simulink library "AFCToolbox2023a"  (R2023a)
settings: Solver=VariableStepAuto  StartTime=0.0  StopTime=10.0  RelTol=1e-3
undefined symbols (not defined in the file or in its folder): AFC5Toolbox_SimuMoudle, AFCToolbox, ax, ay, az, btnSample, C_d, C_dm, C_m, C_t, Control, d, declination_table, dp0, dp1, dp2, dp3, dt, euler_0, g0, I_xyz, inclination_table, J_m, lmd_high, lmd_low, lp_acc_knoise, lp_acc_max, lp_acc_min, lp_acc_seed, lp_GPS_BL_max, lp_GPS_BL_min, lp_GPS_H_max, lp_GPS_H_min, lp_GPS_knoise, lp_GPS_seed, lp_GPS_vel_max, lp_GPS_vel_min, lp_gyro_knoise, lp_gyro_max, lp_gyro_min, lp_gyro_seed, lp_hf_vwind, lp_hs_vwind_interp, lp_kaerorho, lp_kaeroT, lp_kIxyz, lp_kmass, lp_momentx_A0, lp_momentx_Af, lp_momentx_ts, lp_momenty_A0, lp_momenty_Af, lp_momenty_ts, lp_momentz_A0, lp_momentz_Af, lp_momentz_ts, lp_vf_vwind, lp_vs_vwind_interp, lp_vwind_thetax, lp_vwind_thetaz ... (+54)
libraries: $bdroot x104, simulink x75, etargetslib x32, sharedtransform x13, simulink_extras x12, dspstat3 x11, aerolibconvert2 x9, aerolibtransform2 x3, aerolibutil x2, matrix_library x1
(part 6 of 10)

== system AFCToolbox2023a/基础导航算法模型库/ECL EKF/init_state/LLA2NED ==
  note: Vecef2ned
  gps_LLA_rad : Inport
  GPSfixtype : Inport  Port=2
  GPS_Vecef_m/s : Inport  Port=3
  QGC_sensor_reinit : Inport  Port=4
  Angle Conversion1 : aerolibconvert2/Angle Conversion  IU=deg  OU=rad
  Bus Creator : BusCreator  Inputs=3
  Bus Creator2 : BusCreator  Inputs=3
  Bus Selector : BusSelector  OutputSignals=lon_gps,lat_gps
  Bus Selector1 : BusSelector  OutputSignals=lat_gps,lon_gps,H_gps
  Constant1 : Constant  Value=-90
  Constant4 : Constant  Value=0
  Data Type Conversion{,1..3} (4 alike) : DataTypeConversion  OutDataTypeStr=single  SaturateOnIntegerOverflow=off  RndMeth=Floor
  Demux : Demux  Outputs=3
  Demux1 : Demux  Outputs=3
  Demux3 : Demux  Outputs=3
  Detect Increase : simulink/Logic and Bit Operations/Detect Increase  vinit=0.0  OutDataTypeStr=boolean
  Direction Cosine Matrix ECEF to NED : aerolibtransform2/Direction Cosine Matrix ECEF to NED  Commented=on
  Display2 : Display
  Divide1 : Product  Inputs=**  Multiplication=Matrix(*)
  From Workspace22 : FromWorkspace  Commented=on  VariableName=[AFC5_Data.Tim,Pn]  SampleTime=0.01
  From Workspace23 : FromWorkspace  Commented=on  VariableName=[AFC5_Data.Tim,Pe]  SampleTime=0.01
  From Workspace24 : FromWorkspace  Commented=on  VariableName=[AFC5_Data.Tim,Pd]  SampleTime=0.01
  Gain : Gain  Gain=-1
  LLA to ECEF Position : LLA2ECEF  R=6378137
  LLA to ECEF Position1 : LLA2ECEF  R=6378137
  Mux2 : Mux  Inputs=3
  Mux3 : Mux  Commented=on  Inputs=3
  Mux5 : Mux  Inputs=2
  Mux6 : Mux  Inputs=2
  Product : Product  Commented=on  Multiplication=Matrix(*)
  Radians to Degrees{,1..3} (4 alike) : simulink_extras/Transformations/Radians to Degrees
  Radians to Degrees4 : simulink_extras/Transformations/Radians to Degrees  Commented=on
  Rotation Angles to Direction Cosine Matrix : sharedtransform/Rotation Angles to Direction Cosine Matrix  rotationOrder=ZYX  aMode=aMode
  Scope7 : Scope  NumInputPorts=2
  Selector2 : Selector  Commented=on  InputPortWidth=3  IndexOptions=Index vector (dialog)  Indices=[1 2]  OutputSizes=1
  Selector4 : Selector  InputPortWidth=3  IndexOptions=Index vector (dialog)  Indices=[3]  OutputSizes=1
  Sum : Sum  Inputs=|++
  Sum1 : Sum  Inputs=|+-
  initGPSLLA : MATLAB Function  TreatAsAtomicUnit=on
  gpsvNEDout : Outport
  "gpsposNEDout " : Outport  Port=2
  gps_alt_aef : Outport  Port=3
  wires:
  From Workspace24/1 -> Mux3/3
  From Workspace22/1 -> Mux3/1
  From Workspace23/1 -> Mux3/2
  Bus Creator2/1 -> "gpsposNEDout "/1  "data_Pned"
  GPSfixtype/1 -> initGPSLLA/2(GPSfixtype)
  Demux3/3 -> Data Type Conversion2/1  "gpspos_D"
  Demux3/2 -> Data Type Conversion1/1  "gpspos_E"
  Demux3/1 -> Data Type Conversion/1  "gpspos_N"
  Bus Creator/1 -> Bus Selector/1, Bus Selector1/1
  Demux/3 -> Bus Creator/3  "H_gps"
  Demux/2 -> Bus Creator/2  "lon_gps"
  Demux/1 -> Bus Creator/1  "lat_gps"
  Demux1/3 -> LLA to ECEF Position1/2
  Mux6/1 -> LLA to ECEF Position1/1
  Mux5/1 -> LLA to ECEF Position/1
  Gain/1 -> Sum/1
  LLA to ECEF Position1/1 -> Sum1/1
  Constant4/1 -> Mux2/3
  Sum1/1 -> Divide1/2
  Divide1/1 -> Demux3/1
  Demux1/1 -> Radians to Degrees/1
  Rotation Angles to Direction Cosine Matrix/1 -> Divide1/1
  Constant1/1 -> Angle Conversion1/1
  LLA to ECEF Position/1 -> Display2/1, Sum1/2, Selector4/1
  Demux1/2 -> Radians to Degrees1/1
  Sum/1 -> Mux2/2
  Bus Selector/2 -> Gain/1  "<lat_gps>"
  Bus Selector/1 -> Mux2/1  "<lon_gps>"
  Bus Selector1/1 -> Radians to Degrees2/1  "<lat_gps>"
  Bus Selector1/2 -> Radians to Degrees3/1  "<lon_gps>"
  Bus Selector1/3 -> LLA to ECEF Position/2  "<H_gps>"
  Radians to Degrees/1 -> Mux6/1
  Radians to Degrees1/1 -> Mux6/2
  QGC_sensor_reinit/1 -> Detect Increase/1
  Data Type Conversion/1 -> Bus Creator2/1  "gpspos_N"
  Data Type Conversion1/1 -> Bus Creator2/2  "gpspos_E"
  Angle Conversion1/1 -> Sum/2
  Radians to Degrees2/1 -> Mux5/1
  Radians to Degrees3/1 -> Mux5/2
  GPS_Vecef_m/s/1 -> Data Type Conversion3/1
  Direction Cosine Matrix ECEF to NED/1 -> Product/1
  Selector2/1 -> Radians to Degrees4/1
  Radians to Degrees4/1 -> Direction Cosine Matrix ECEF to NED/1
  Data Type Conversion3/1 -> gpsvNEDout/1
  Detect Increase/1 -> initGPSLLA/1(QGCinitflag)
  initGPSLLA/1(gpsLLA0_rad) -> Demux/1
  Selector4/1 -> Scope7/2
  Mux2/1 -> Rotation Angles to Direction Cosine Matrix/1
  gps_LLA_rad/1 -> Selector2/1, Demux1/1, initGPSLLA/3(gps_LLA_rad)
  Data Type Conversion2/1 -> Bus Creator2/3  "gpspos_D"

== system AFCToolbox2023a/基础导航算法模型库/ECL EKF/init_state/State_mag1 ==
  mag : Inport
  gps_LLA_rad : Inport  Port=2
  states : Inport  Port=3
  Atan2 : Trigonometry  Operator=atan2
  Bus Creator : BusCreator  Inputs=5
  Constant1 : Constant
  Constant2 : Constant  Value=0
  Data Type Conversion1 : DataTypeConversion  OutDataTypeStr=double  SaturateOnIntegerOverflow=off  RndMeth=Floor
  Data Type Conversion2 : DataTypeConversion  OutDataTypeStr=double  SaturateOnIntegerOverflow=off  RndMeth=Floor
  Data Type Conversion3 : DataTypeConversion  OutDataTypeStr=double  SaturateOnIntegerOverflow=off  RndMeth=Floor
  Demux : Demux  Outputs=3
  Demux2 : Demux  Outputs=3
  Detect Increase : simulink/Logic and Bit Operations/Detect Increase  vinit=0.0  OutDataTypeStr=boolean
  Digital Clock : DigitalClock  SampleTime=-1
  Display : Display
  Display1 : Display
  Display2 : Display
  Math Function2 : Math  Commented=on  Operator=transpose  SignedPower=on
  Memory : Memory  InheritSampleTime=on
  Mux2 : Mux  Inputs=3
  Quaternions to Direction Cosine Matrix : sharedtransform/Quaternions to  Direction Cosine Matrix  Commented=on  aMode=aMode
      settings: LibrarySourceBlock=|
      | aerolibtransform2/Quaternions to
      | Direction Cosine Matrix
  Radians to Degrees : simulink_extras/Transformations/Radians to Degrees
  Scope{1..6} (6 alike) : Scope
  Selector1 : Selector  Commented=on  InputPortWidth=24  IndexOptions=Index vector (dialog)  Indices=[1,2,3,4]  OutputSizes=1
  Subsystem : Subsystem
  Subsystem1 : Subsystem  Commented=on  mask{declination_table=declination_table, inclination_table=inclination_table, strength_table=strength_table}
      mask prompts: declination_table "Declination Lookup Table"; inclination_table "Magnitude Lookup Table"; strength_table "Inclination Lookup Table"
      mask DialogControl ParameterGroupVar Prompt: 参数
  Switch : Switch  Criteria=u2 > Threshold  SaturateOnIntegerOverflow=off  InputSameDT=off
  Switch2 : Switch  Threshold=1  SaturateOnIntegerOverflow=off  InputSameDT=off
  Terminator : Terminator
  Terminator1 : Terminator
  Zero-Order Hold : ZeroOrderHold  SampleTime=-1
  calculate_synthetic_mag_z_measurement : Subsystem  Commented=on
  initMag1 : MATLAB Function  Commented=on  TreatAsAtomicUnit=on
  mag_lpf : Subsystem
  init_MagB : Outport
  magdata : Outport  Port=2
  wires:
  Radians to Degrees/1 -> Scope6/1
  Atan2/1 -> Radians to Degrees/1
  Bus Creator/1 -> magdata/1
  gps_LLA_rad/1 -> Demux/1
  Demux/1 -> Scope2/1, Subsystem1/1(lat_rad)
  Demux/2 -> Subsystem1/2(lon_rad)
  Demux/3 -> Terminator/1
  Demux2/1 -> Mux2/1, Atan2/2
  mag/1 -> Scope5/1, Bus Creator/2, Demux2/1, calculate_synthetic_mag_z_measurement/1(measMag), Zero-Order Hold/1, Display1/1, mag_lpf/1(Mag_Data)  "measMag"
  Demux2/2 -> Mux2/2, Atan2/1
  Subsystem1/1(mag_declination_gps) -> Scope1/1, Data Type Conversion2/1  "mag_declination_gps"
  Subsystem1/2(mag_inclination_gps) -> Data Type Conversion1/1, Scope3/1  "mag_inclination_gps"
  Subsystem1/3(mag_strength_gps) -> Data Type Conversion3/1  "mag_strength_gps"
  calculate_synthetic_mag_z_measurement/1(mag_z_body_pred) -> Mux2/3
  Quaternions to Direction Cosine Matrix/1 -> Math Function2/1
  Demux2/3 -> Terminator1/1
  Data Type Conversion2/1 -> Display/1, calculate_synthetic_mag_z_measurement/2(_mag_declination_gps), Bus Creator/3  "mag_declination_gps"
  Data Type Conversion1/1 -> calculate_synthetic_mag_z_measurement/3(_mag_inclination_gps), Bus Creator/4  "mag_inclination_gps"
  Data Type Conversion3/1 -> calculate_synthetic_mag_z_measurement/4(_mag_strength_gps), Bus Creator/5  "mag_strength_gps"
  states/1 -> Selector1/1
  Selector1/1 -> Quaternions to Direction Cosine Matrix/1
  Constant2/1 -> Switch/3
  Digital Clock/1 -> Switch/2
  Constant1/1 -> Switch/1
  Switch/1 -> Detect Increase/1
  Detect Increase/1 -> Switch2/2
  Zero-Order Hold/1 -> Switch2/1, Memory/1, Display2/1, init_MagB/1, Bus Creator/1, Subsystem/1(data)  "init_MagB"
  Memory/1 -> Switch2/3

== system AFCToolbox2023a/SimuMoudle/Forces & Moments1/Moments/Disturb/Dist Mx ==
  N : Inport
  Step2 : Step  Time=ts_0  Before=A0  After=Af
  Sum : Sum  Inputs=|++
  D : Outport
  wires:
  Sum/1 -> D/1
  N/1 -> Sum/1
  Step2/1 -> Sum/2

== system AFCToolbox2023a/SimuMoudle/Forces & Moments1/Moments/Disturb/Dist My ==
  N : Inport
  Step2 : Step  Time=ts_0  Before=A0  After=Af
  Sum : Sum  Inputs=|++
  D : Outport
  wires:
  Step2/1 -> Sum/2
  N/1 -> Sum/1
  Sum/1 -> D/1

== system AFCToolbox2023a/SimuMoudle/Forces & Moments1/Moments/Disturb/Dist Mz ==
  N : Inport
  Step2 : Step  Time=ts_0  Before=A0  After=Af
  Sum : Sum  Inputs=|++
  D : Outport
  wires:
  Sum/1 -> D/1
  N/1 -> Sum/1
  Step2/1 -> Sum/2

== system AFCToolbox2023a/SimuMoudle/Forces & Moments1/Parameters/Air Parameter1/Air Model ==
  note: rho
  v : Inport
  h (km) : Inport  Port=2
  1/2 : Constant  Value=0.5
  Gain lp_kaeroT : Gain  Gain=lp_kaeroT
  Gain lp_kaerorho : Gain  Gain=lp_kaerorho
  H : Subsystem
      mask Display: disp('h --> H')
  Math Function : Math  Operator=sqrt  SignedPower=on
  Math Function1 : Math  Operator=pow  SignedPower=on
  Math Function2 : Math  Operator=pow  SignedPower=on
  PSL : Constant  Value=101325
  Pressure xishu : Subsystem
  Product : Product  Inputs=/*  SaturateOnIntegerOverflow=on  OutDataTypeStr=Inherit: Same as first input
  Product1 : Product  RndMeth=Zero
  Product2 : Product  Inputs=3  RndMeth=Zero
  Product3 : Product  Inputs=4  RndMeth=Zero
  Product4 : Product  Inputs=3  RndMeth=Zero
  T : Subsystem
  T xishu : Subsystem
  W : Subsystem
  W zhishu : Subsystem
  W zhishu1 : Subsystem
  constant2 : Constant  Value=20.0468
  rho xishu : Subsystem
  rhoSL : Constant  Value=1.225
  dongYaTou : Outport
  Mach : Outport  Port=2
  Pressure : Outport  Port=3
  wires:
  Product4/1 -> Pressure/1
  PSL/1 -> Product4/3
  Math Function2/1 -> Product4/1
  Pressure xishu/1(xishu) -> Product4/2
  W zhishu1/1(zhishu) -> Math Function2/2
  Gain lp_kaerorho/1 -> Product3/4
  Gain lp_kaeroT/1 -> Math Function/1
  v/1 -> Product3/1, Product/2, Product3/2
  Product/1 -> Mach/1
  Product1/1 -> Product/1
  1/2/1 -> Product3/3
  T/1(T) -> Gain lp_kaeroT/1
  h (km)/1 -> H/1(h), T/1(Z), Pressure xishu/1(Z), W zhishu1/1(Z), rho xishu/1(Z), W zhishu/1(Z), W/2(Z), T xishu/1(Z)
  H/1(H) -> Pressure xishu/2(H), W/1(H)
  W zhishu/1(zhishu) -> Math Function1/2
  Product3/1 -> dongYaTou/1
  Product2/1 -> Gain lp_kaerorho/1
  rhoSL/1 -> Product2/3
  rho xishu/1(xishu) -> Product2/2
  Math Function1/1 -> Product2/1
  W/1(W) -> Math Function2/1, Math Function1/1, T/3(W)
  T xishu/1(T xishu) -> T/2(T xishu)
  constant2/1 -> Product1/2
  Math Function/1 -> Product1/1

== system AFCToolbox2023a/SimuMoudle/Forces & Moments1/Parameters/Wind Velocity/Vector ==
  abs : Inport
  thetaz : Inport  Port=2
  thetax : Inport  Port=3
  Mux : Mux  Inputs=3
  Selector : Selector  InputPortWidth=3  IndexOptions=Index vector (dialog)  Indices=[3 2 1]  OutputSizes=1
  sin thetax cos thetax : Trigonometry  Operator=sincos
  sin thetaz cos thetaz : Trigonometry  Operator=sincos
  vwind cos z : Product  RndMeth=Zero
  vwind sin z : Product  RndMeth=Zero
  vwind xy cos x : Product  RndMeth=Zero
  vwind xy sin x : Product  RndMeth=Zero
  xyz : Outport
  wires:
  abs/1 -> vwind cos z/1, vwind sin z/1
  sin thetaz cos thetaz/1 -> vwind sin z/2
  sin thetaz cos thetaz/2 -> vwind cos z/2
  vwind sin z/1 -> Mux/1
  sin thetax cos thetax/1 -> vwind xy sin x/2
  sin thetax cos thetax/2 -> vwind xy cos x/2
  vwind cos z/1 -> vwind xy cos x/1, vwind xy sin x/1
  vwind xy cos x/1 -> Mux/3
  vwind xy sin x/1 -> Mux/2
  Mux/1 -> Selector/1
  thetaz/1 -> sin thetaz cos thetaz/1
  Selector/1 -> xyz/1
  thetax/1 -> sin thetax cos thetax/1

== system AFCToolbox2023a/SimuMoudle/Position-Control/Consistent formation control /一致性控制——F1/Subsystem1 ==
  Constant : Constant  Value=0.01
  MATLAB Function : MATLAB Function  TreatAsAtomicUnit=on
  Mux : Mux  Inputs=3
  Ramp : simulink/Sources/Ramp  slope=1  start=0  InitialOutput=0
  wxyz : Outport
  wires:
  Mux/1 -> wxyz/1
  MATLAB Function/2(wy) -> Mux/2, Mux/3
  MATLAB Function/1(wx) -> Mux/1
  Constant/1 -> MATLAB Function/2(dt)
  Ramp/1 -> MATLAB Function/1(i)

== system AFCToolbox2023a/SimuMoudle/Position-Control/Consistent formation control /一致性控制——F2/Subsystem2 ==
  Constant : Constant  Value=0.01
  MATLAB Function : MATLAB Function  TreatAsAtomicUnit=on
  Mux : Mux  Inputs=3
  Ramp : simulink/Sources/Ramp  slope=1  start=0  InitialOutput=0
  wxyz : Outport
  wires:
  Mux/1 -> wxyz/1
  MATLAB Function/2(wy) -> Mux/2, Mux/3
  MATLAB Function/1(wx) -> Mux/1
  Constant/1 -> MATLAB Function/2(dt)
  Ramp/1 -> MATLAB Function/1(i)

== system AFCToolbox2023a/SimuMoudle/Position-Control/Consistent formation control /一致性控制——F3/Subsystem1 ==
  Constant : Constant  Value=0.01
  MATLAB Function : MATLAB Function  TreatAsAtomicUnit=on
  Mux : Mux  Inputs=3
  Ramp : simulink/Sources/Ramp  slope=1  start=0  InitialOutput=0
  wxyz : Outport
  wires:
  Mux/1 -> wxyz/1
  MATLAB Function/2(wy) -> Mux/2, Mux/3
  MATLAB Function/1(wx) -> Mux/1
  Constant/1 -> MATLAB Function/2(dt)
  Ramp/1 -> MATLAB Function/1(i)

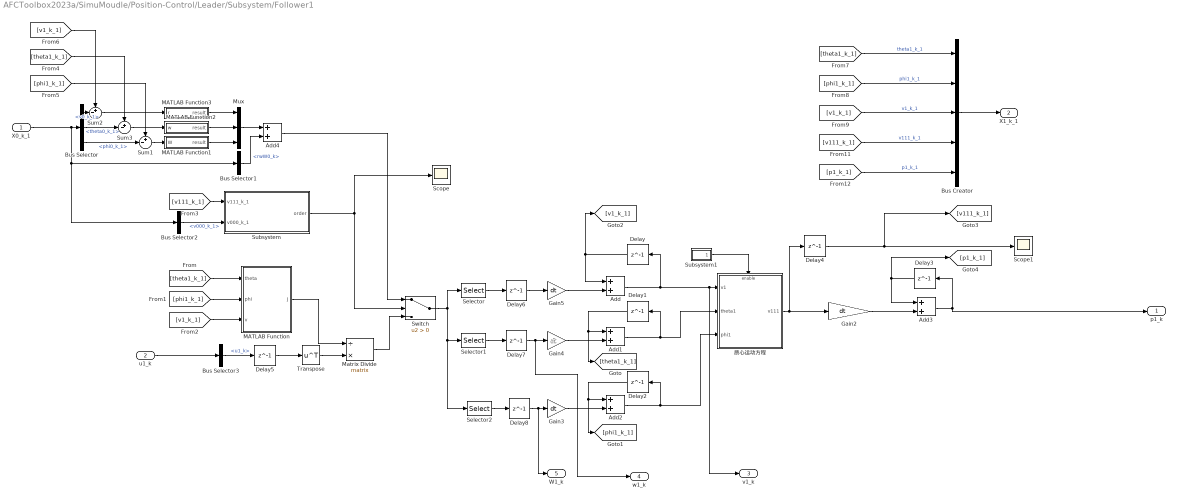
== system AFCToolbox2023a/SimuMoudle/Position-Control/Leader/Subsystem/Follower1 ==
  note: dt
  X0_k_1 : Inport
  u1_k : Inport  Port=2
  Add{,1..4} (5 alike) : Sum
  Bus Creator : BusCreator  Inputs=5
  Bus Selector : BusSelector  OutputSignals=v0_k_1,theta0_k_1,phi0_k_1
  Bus Selector1 : BusSelector  OutputSignals=rwW0_k
  Bus Selector2 : BusSelector  OutputSignals=v000_k_1
  Bus Selector3 : BusSelector  OutputSignals=u1_k
  Delay : Delay  DelayLength=1  InitialCondition=v1
  Delay1 : Delay  DelayLength=1  InitialCondition=theta1
  Delay2 : Delay  DelayLength=1  InitialCondition=phi1
  Delay3 : Delay  DelayLength=1  InitialCondition=p1
  Delay4 : Delay  DelayLength=1  InitialCondition=v111
  Delay5 : Delay  DelayLength=1  InitialCondition=u1
  Delay6 : Delay  DelayLength=1  InitialCondition=r1
  Delay7 : Delay  DelayLength=1  InitialCondition=w1
  Delay8 : Delay  DelayLength=1  InitialCondition=W1
  Gain{2..5} (4 alike) : Gain  Gain=dt
  MATLAB Function : MATLAB Function  TreatAsAtomicUnit=on
  MATLAB Function1 : MATLAB Function  TreatAsAtomicUnit=on
  MATLAB Function2 : MATLAB Function  TreatAsAtomicUnit=on
  MATLAB Function3 : MATLAB Function  TreatAsAtomicUnit=on
  Matrix Divide : Product  Inputs=/*  Multiplication=Matrix(*)
  Mux : Mux  Inputs=3
  Scope : Scope
  Scope1 : Scope
  Selector : Selector  InputPortWidth=3  IndexOptions=Index vector (dialog)  Indices=[1]  OutputSizes=1
  Selector1 : Selector  InputPortWidth=3  IndexOptions=Index vector (dialog)  Indices=[2]  OutputSizes=1
  Selector2 : Selector  InputPortWidth=3  IndexOptions=Index vector (dialog)  Indices=[3]  OutputSizes=1
  Subsystem : Subsystem
  Subsystem1 : Subsystem
  Sum1 : Sum  Inputs=+-|
  Sum2 : Sum  Inputs=+-|
  Sum3 : Sum  Inputs=+-|
  Switch : Switch  Criteria=u2 > Threshold  SaturateOnIntegerOverflow=off  InputSameDT=off
  Transpose : Math  Operator=transpose
  质心运动方程 : Subsystem
  p1_k : Outport
  X1_k_1 : Outport  Port=2
  v1_k : Outport  Port=3
  w1_k : Outport  Port=4
  W1_k : Outport  Port=5
  wires:
  Subsystem1/1(Out1) -> 质心运动方程/Enable
  Add3/1 -> Delay3/1, p1_k/1
  Delay1/1 -> Add1/1, [theta1_k_1]
  Transpose/1 -> Matrix Divide/2
  Bus Selector3/1 -> Delay5/1  "<u1_k>"
  Delay4/1 -> Scope1/1, [v111_k_1]
  Delay8/1 -> Gain3/1, W1_k/1
  Delay7/1 -> Gain4/1, w1_k/1
  Delay6/1 -> Gain5/1
  Add4/1 -> Switch/1
  Delay5/1 -> Transpose/1
  [theta1_k_1] -> Bus Creator/1  "theta1_k_1"
  [phi1_k_1] -> Bus Creator/2  "phi1_k_1"
  Bus Creator/1 -> X1_k_1/1
  [v1_k_1] -> Bus Creator/3  "v1_k_1"
  [p1_k_1] -> Bus Creator/5  "p1_k_1"
  [v111_k_1] -> Bus Creator/4  "v111_k_1"
  [v1_k_1] -> Sum2/1
  [phi1_k_1] -> Sum1/1
  [theta1_k_1] -> Sum3/1
  Sum1/1 -> MATLAB Function1/1(W)
  Sum2/1 -> MATLAB Function3/1(r)
  Bus Selector/1 -> Sum2/2  "<v0_k_1>"
  Bus Selector/3 -> Sum1/2  "<phi0_k_1>"
  Sum3/1 -> MATLAB Function2/1(w)
  Bus Selector/2 -> Sum3/2  "<theta0_k_1>"
  Mux/1 -> Add4/1
  MATLAB Function3/1(result) -> Mux/1
  MATLAB Function1/1(result) -> Mux/3
  MATLAB Function2/1(result) -> Mux/2
  Bus Selector1/1 -> Add4/2  "<rwW0_k>"
  X0_k_1/1 -> Bus Selector/1, Bus Selector1/1, Bus Selector2/1
  Bus Selector2/1 -> Subsystem/2(v000_k_1)  "<v000_k_1>"
  [v111_k_1] -> Subsystem/1(v111_k_1)
  质心运动方程/1(v111) -> Gain2/1, Delay4/1
  Matrix Divide/1 -> Switch/3
  Subsystem/1(order) -> Scope/1, Switch/2
  Selector2/1 -> Delay8/1
  Selector1/1 -> Delay7/1
  Selector/1 -> Delay6/1
  u1_k/1 -> Bus Selector3/1
  MATLAB Function/1(J) -> Matrix Divide/1
  Gain5/1 -> Add/2
  Add/1 -> Delay/1, 质心运动方程/1(v1), v1_k/1
  Delay/1 -> [v1_k_1], Add/1
  Add1/1 -> Delay1/1, 质心运动方程/2(theta1)
  Add2/1 -> Delay2/1, 质心运动方程/3(phi1)
  Delay2/1 -> Add2/1, [phi1_k_1]
  Gain2/1 -> Add3/2
  Delay3/1 -> [p1_k_1], Add3/1
  Switch/1 -> Selector/1, Selector1/1, Selector2/1
  Gain3/1 -> Add2/2
  Gain4/1 -> Add1/2
  [theta1_k_1] -> MATLAB Function/1(theta)
  [phi1_k_1] -> MATLAB Function/2(phi)
  [v1_k_1] -> MATLAB Function/3(v)

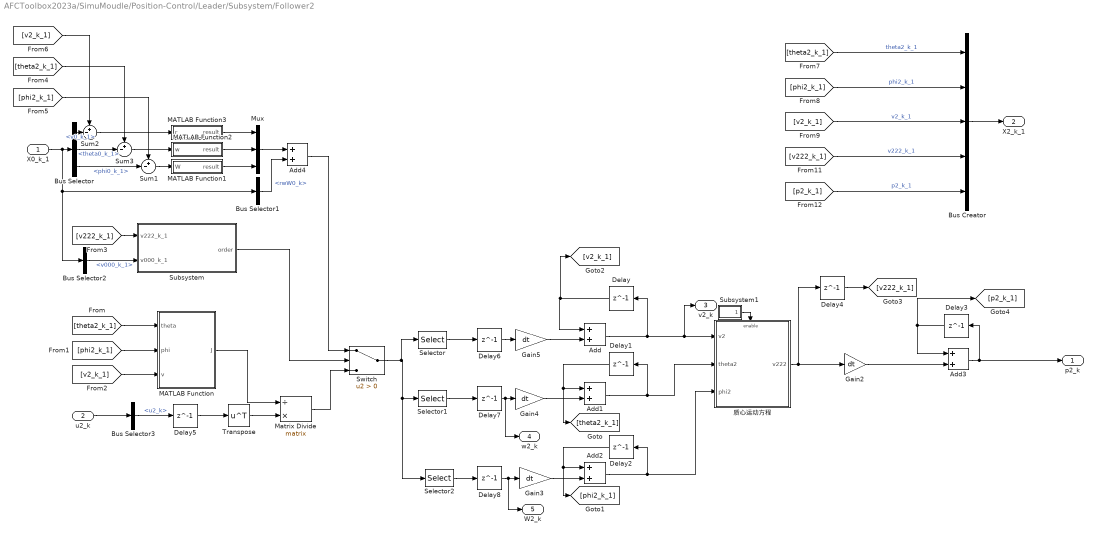
== system AFCToolbox2023a/SimuMoudle/Position-Control/Leader/Subsystem/Follower2 ==
  X0_k_1 : Inport
  u2_k : Inport  Port=2
  Add{,1..4} (5 alike) : Sum
  Bus Creator : BusCreator  Inputs=5
  Bus Selector : BusSelector  OutputSignals=v0_k_1,theta0_k_1,phi0_k_1
  Bus Selector1 : BusSelector  OutputSignals=rwW0_k
  Bus Selector2 : BusSelector  OutputSignals=v000_k_1
  Bus Selector3 : BusSelector  OutputSignals=u2_k
  Delay : Delay  DelayLength=1  InitialCondition=v2
  Delay1 : Delay  DelayLength=1  InitialCondition=theta2
  Delay2 : Delay  DelayLength=1  InitialCondition=phi2
  Delay3 : Delay  DelayLength=1  InitialCondition=p2
  Delay4 : Delay  DelayLength=1  InitialCondition=v222
  Delay5 : Delay  DelayLength=1  InitialCondition=u2
  Delay6 : Delay  DelayLength=1  InitialCondition=w2
  Delay7 : Delay  DelayLength=1  InitialCondition=W2
  Delay8 : Delay  DelayLength=1  InitialCondition=r2
  Gain{2..5} (4 alike) : Gain  Gain=dt
  MATLAB Function : MATLAB Function  TreatAsAtomicUnit=on
  MATLAB Function1 : MATLAB Function  TreatAsAtomicUnit=on
  MATLAB Function2 : MATLAB Function  TreatAsAtomicUnit=on
  MATLAB Function3 : MATLAB Function  TreatAsAtomicUnit=on
  Matrix Divide : Product  Inputs=/*  Multiplication=Matrix(*)
  Mux : Mux  Inputs=3
  Selector : Selector  InputPortWidth=3  IndexOptions=Index vector (dialog)  Indices=[1]  OutputSizes=1
  Selector1 : Selector  InputPortWidth=3  IndexOptions=Index vector (dialog)  Indices=[2]  OutputSizes=1
  Selector2 : Selector  InputPortWidth=3  IndexOptions=Index vector (dialog)  Indices=[3]  OutputSizes=1
  Subsystem : Subsystem
  Subsystem1 : Subsystem
  Sum1 : Sum  Inputs=+-|
  Sum2 : Sum  Inputs=+-|
  Sum3 : Sum  Inputs=+-|
  Switch : Switch  Criteria=u2 > Threshold  SaturateOnIntegerOverflow=off  InputSameDT=off
  Transpose : Math  Operator=transpose
  质心运动方程 : Subsystem
  p2_k : Outport
  X2_k_1 : Outport  Port=2
  v2_k : Outport  Port=3
  w2_k : Outport  Port=4
  W2_k : Outport  Port=5
  wires:
  Subsystem1/1(Out1) -> 质心运动方程/Enable
  Delay4/1 -> [v222_k_1]
  Delay3/1 -> Add3/1, [p2_k_1]
  Add3/1 -> p2_k/1, Delay3/1
  Transpose/1 -> Matrix Divide/2
  Bus Selector3/1 -> Delay5/1  "<u2_k>"
  Delay8/1 -> Gain3/1, W2_k/1
  Delay7/1 -> Gain4/1, w2_k/1
  Delay6/1 -> Gain5/1
  Delay5/1 -> Transpose/1
  [v2_k_1] -> MATLAB Function/3(v)
  [phi2_k_1] -> MATLAB Function/2(phi)
  [theta2_k_1] -> MATLAB Function/1(theta)
  Gain4/1 -> Add1/2
  Gain3/1 -> Add2/2
  Switch/1 -> Selector2/1, Selector1/1, Selector/1
  Gain2/1 -> Add3/2
  质心运动方程/1(v222) -> Delay4/1, Gain2/1
  Delay2/1 -> Add2/1, [phi2_k_1]
  Add2/1 -> Delay2/1, 质心运动方程/3(phi2)
  Add1/1 -> Delay1/1, 质心运动方程/2(theta2)
  Delay1/1 -> Add1/1, [theta2_k_1]
  Delay/1 -> Add/1, [v2_k_1]
  Add/1 -> 质心运动方程/1(v2), v2_k/1, Delay/1
  Gain5/1 -> Add/2
  MATLAB Function/1(J) -> Matrix Divide/1
  u2_k/1 -> Bus Selector3/1
  Selector/1 -> Delay6/1
  Selector1/1 -> Delay7/1
  Selector2/1 -> Delay8/1
  Add4/1 -> Switch/1
  Subsystem/1(order) -> Switch/2
  Matrix Divide/1 -> Switch/3
  [v222_k_1] -> Subsystem/1(v222_k_1)
  Bus Selector2/1 -> Subsystem/2(v000_k_1)  "<v000_k_1>"
  X0_k_1/1 -> Bus Selector2/1, Bus Selector1/1, Bus Selector/1
  Bus Selector1/1 -> Add4/2  "<rwW0_k>"
  MATLAB Function2/1(result) -> Mux/2
  MATLAB Function1/1(result) -> Mux/3
  MATLAB Function3/1(result) -> Mux/1
  Mux/1 -> Add4/1
  Bus Selector/2 -> Sum3/2  "<theta0_k_1>"
  Sum3/1 -> MATLAB Function2/1(w)
  Bus Selector/3 -> Sum1/2  "<phi0_k_1>"
  Bus Selector/1 -> Sum2/2  "<v0_k_1>"
  Sum2/1 -> MATLAB Function3/1(r)
  Sum1/1 -> MATLAB Function1/1(W)
  [theta2_k_1] -> Sum3/1
  [phi2_k_1] -> Sum1/1
  [v2_k_1] -> Sum2/1
  [v222_k_1] -> Bus Creator/4  "v222_k_1"
  [p2_k_1] -> Bus Creator/5  "p2_k_1"
  [v2_k_1] -> Bus Creator/3  "v2_k_1"
  Bus Creator/1 -> X2_k_1/1
  [phi2_k_1] -> Bus Creator/2  "phi2_k_1"
  [theta2_k_1] -> Bus Creator/1  "theta2_k_1"

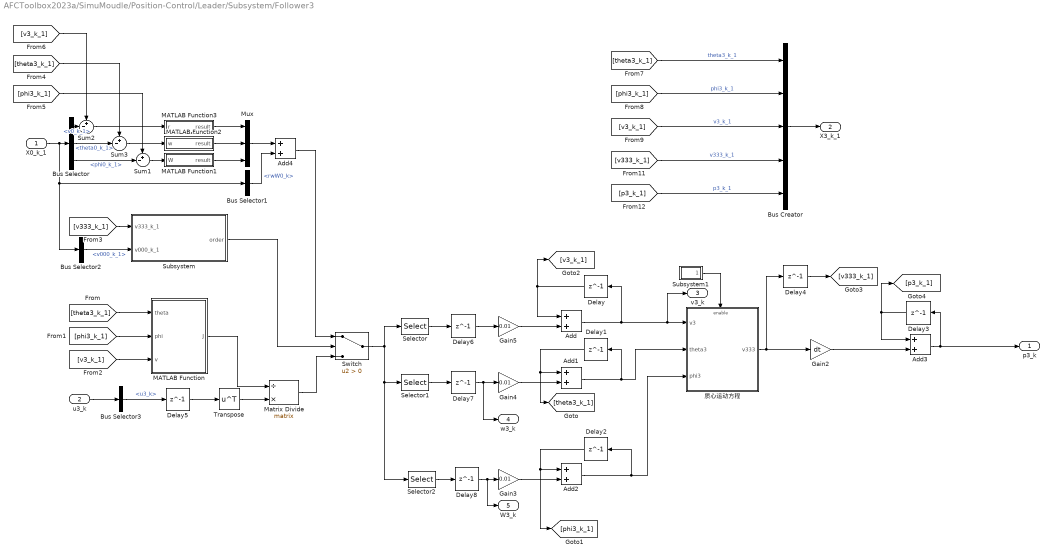
== system AFCToolbox2023a/SimuMoudle/Position-Control/Leader/Subsystem/Follower3 ==
  X0_k_1 : Inport
  u3_k : Inport  Port=2
  Add{,1..4} (5 alike) : Sum
  Bus Creator : BusCreator  Inputs=5
  Bus Selector : BusSelector  OutputSignals=v0_k_1,theta0_k_1,phi0_k_1
  Bus Selector1 : BusSelector  OutputSignals=rwW0_k
  Bus Selector2 : BusSelector  OutputSignals=v000_k_1
  Bus Selector3 : BusSelector  OutputSignals=u3_k
  Delay : Delay  DelayLength=1  InitialCondition=v3
  Delay1 : Delay  DelayLength=1  InitialCondition=theta3
  Delay2 : Delay  DelayLength=1  InitialCondition=phi3
  Delay3 : Delay  DelayLength=1  InitialCondition=p3
  Delay4 : Delay  DelayLength=1  InitialCondition=v333
  Delay5 : Delay  DelayLength=1  InitialCondition=u3
  Delay6 : Delay  DelayLength=1  InitialCondition=r3
  Delay7 : Delay  DelayLength=1  InitialCondition=w3
  Delay8 : Delay  DelayLength=1  InitialCondition=W3
  Gain2 : Gain  Gain=dt
  Gain3 : Gain  Gain=0.01
  Gain4 : Gain  Gain=0.01
  Gain5 : Gain  Gain=0.01
  MATLAB Function : MATLAB Function  TreatAsAtomicUnit=on
  MATLAB Function1 : MATLAB Function  TreatAsAtomicUnit=on
  MATLAB Function2 : MATLAB Function  TreatAsAtomicUnit=on
  MATLAB Function3 : MATLAB Function  TreatAsAtomicUnit=on
  Matrix Divide : Product  Inputs=/*  Multiplication=Matrix(*)
  Mux : Mux  Inputs=3
  Selector : Selector  InputPortWidth=3  IndexOptions=Index vector (dialog)  Indices=[1]  OutputSizes=1
  Selector1 : Selector  InputPortWidth=3  IndexOptions=Index vector (dialog)  Indices=[2]  OutputSizes=1
  Selector2 : Selector  InputPortWidth=3  IndexOptions=Index vector (dialog)  Indices=[3]  OutputSizes=1
  Subsystem : Subsystem
  Subsystem1 : Subsystem
  Sum1 : Sum  Inputs=+-|
  Sum2 : Sum  Inputs=+-|
  Sum3 : Sum  Inputs=+-|
  Switch : Switch  Criteria=u2 > Threshold  SaturateOnIntegerOverflow=off  InputSameDT=off
  Transpose : Math  Operator=transpose
  质心运动方程 : Subsystem
  p3_k : Outport
  X3_k_1 : Outport  Port=2
  v3_k : Outport  Port=3
  w3_k : Outport  Port=4
  W3_k : Outport  Port=5
  wires:
  Subsystem1/1(Out1) -> 质心运动方程/Enable
  Delay4/1 -> [v333_k_1]
  Add3/1 -> Delay3/1, p3_k/1
  Transpose/1 -> Matrix Divide/2
  Bus Selector3/1 -> Delay5/1  "<u3_k>"
  Delay5/1 -> Transpose/1
  Delay8/1 -> Gain3/1, W3_k/1
  Delay7/1 -> Gain4/1, w3_k/1
  Delay6/1 -> Gain5/1
  [theta3_k_1] -> Bus Creator/1  "theta3_k_1"
  [phi3_k_1] -> Bus Creator/2  "phi3_k_1"
  Bus Creator/1 -> X3_k_1/1
  [v3_k_1] -> Bus Creator/3  "v3_k_1"
  [p3_k_1] -> Bus Creator/5  "p3_k_1"
  [v333_k_1] -> Bus Creator/4  "v333_k_1"
  [v3_k_1] -> Sum2/1
  [phi3_k_1] -> Sum1/1
  [theta3_k_1] -> Sum3/1
  Sum1/1 -> MATLAB Function1/1(W)
  Sum2/1 -> MATLAB Function3/1(r)
  Bus Selector/1 -> Sum2/2  "<v0_k_1>"
  Bus Selector/3 -> Sum1/2  "<phi0_k_1>"
  Sum3/1 -> MATLAB Function2/1(w)
  Bus Selector/2 -> Sum3/2  "<theta0_k_1>"
  Mux/1 -> Add4/1
  MATLAB Function3/1(result) -> Mux/1
  MATLAB Function1/1(result) -> Mux/3
  MATLAB Function2/1(result) -> Mux/2
  Bus Selector1/1 -> Add4/2  "<rwW0_k>"
  X0_k_1/1 -> Bus Selector/1, Bus Selector1/1, Bus Selector2/1
  Bus Selector2/1 -> Subsystem/2(v000_k_1)  "<v000_k_1>"
  [v333_k_1] -> Subsystem/1(v333_k_1)
  Matrix Divide/1 -> Switch/3
  Subsystem/1(order) -> Switch/2
  Add4/1 -> Switch/1
  Selector2/1 -> Delay8/1
  Selector1/1 -> Delay7/1
  Selector/1 -> Delay6/1
  u3_k/1 -> Bus Selector3/1
  MATLAB Function/1(J) -> Matrix Divide/1
  Gain5/1 -> Add/2
  Add/1 -> 质心运动方程/1(v3), v3_k/1, Delay/1
  Delay/1 -> [v3_k_1], Add/1
  Delay1/1 -> [theta3_k_1], Add1/1
  Add1/1 -> Delay1/1, 质心运动方程/2(theta3)
  Add2/1 -> 质心运动方程/3(phi3), Delay2/1
  Delay2/1 -> Add2/1, [phi3_k_1]
  质心运动方程/1(v333) -> Gain2/1, Delay4/1
  Gain2/1 -> Add3/2
  Delay3/1 -> Add3/1, [p3_k_1]
  Switch/1 -> Selector/1, Selector2/1, Selector1/1
  Gain3/1 -> Add2/2
  Gain4/1 -> Add1/2
  [theta3_k_1] -> MATLAB Function/1(theta)
  [phi3_k_1] -> MATLAB Function/2(phi)
  [v3_k_1] -> MATLAB Function/3(v)

== system AFCToolbox2023a/SimuMoudle/SimuGps/LLA model/Subsystem1/LLA2NED ==
  LLA0 : Inport
  LLA : Inport  Port=2
  Angle Conversion2 : aerolibconvert2/Angle Conversion  IU=deg  OU=rad
  Angle Conversion3 : aerolibconvert2/Angle Conversion  IU=deg  OU=rad
  Bus Selector : BusSelector  OutputSignals=lon,lat
  Bus Selector1 : BusSelector  OutputSignals=lat,lon,alt
  Bus Selector5 : BusSelector  OutputSignals=lat,lon,alt
  Constant1 : Constant  Value=-90
  Constant4 : Constant  Value=0
  Demux3 : Demux  Outputs=3
  Divide1 : Product  Inputs=**  Multiplication=Matrix(*)
  Gain : Gain  Gain=-1
  Gain1 : Gain  Gain=-1
  LLA to ECEF Position : LLA2ECEF  R=6378137
  LLA to ECEF Position1 : LLA2ECEF  R=6378137
  Mux : Mux  Inputs=3
  Mux2 : Mux  Inputs=3
  Mux5 : Mux  Inputs=2
  Mux6 : Mux  Inputs=2
  Radians to Degrees : simulink_extras/Transformations/Radians to Degrees
  Radians to Degrees1 : simulink_extras/Transformations/Radians to Degrees
  Rotation Angles to Direction Cosine Matrix : sharedtransform/Rotation Angles to Direction Cosine Matrix  rotationOrder=ZYX  aMode=aMode
  Sum : Sum  Inputs=|++
  Sum1 : Sum  Inputs=|+-
  "sensorout " : Outport
  wires:
  Gain1/1 -> Mux/2
  Demux3/2 -> Mux/3  "Yeast"
  Demux3/3 -> Gain1/1
  Demux3/1 -> Mux/1  "Xnorth"
  Radians to Degrees1/1 -> Mux6/2
  Radians to Degrees/1 -> Mux6/1
  LLA/1 -> Bus Selector5/1
  Mux/1 -> "sensorout "/1
  Bus Selector1/3 -> LLA to ECEF Position/2  "<alt>"
  Bus Selector1/2 -> Mux5/2  "<lon>"
  Bus Selector1/1 -> Mux5/1  "<lat>"
  Bus Selector/1 -> Angle Conversion2/1  "<lon>"
  Bus Selector/2 -> Gain/1  "<lat>"
  Angle Conversion3/1 -> Mux2/2
  Bus Selector5/2 -> Radians to Degrees1/1  "<lon>"
  Angle Conversion2/1 -> Mux2/1
  LLA to ECEF Position/1 -> Sum1/2
  Constant1/1 -> Sum/2
  [M_ecef2ned] -> Divide1/1
  Rotation Angles to Direction Cosine Matrix/1 -> [M_ecef2ned]
  Mux2/1 -> Rotation Angles to Direction Cosine Matrix/1
  Bus Selector5/1 -> Radians to Degrees/1  "<lat>"
  Divide1/1 -> Demux3/1
  [LLA0] -> Bus Selector/1
  [LLA0] -> Bus Selector1/1
  Sum1/1 -> Divide1/2
  Constant4/1 -> Mux2/3
  LLA to ECEF Position1/1 -> Sum1/1
  Gain/1 -> Sum/1
  Mux5/1 -> LLA to ECEF Position/1
  Mux6/1 -> LLA to ECEF Position1/1
  LLA0/1 -> [LLA0]
  Sum/1 -> Angle Conversion3/1
  Bus Selector5/3 -> LLA to ECEF Position1/2  "<alt>"

== system AFCToolbox2023a/SimuMoudle/SimuICM/acclerate  model2/Subsystem/bias & noise x1 ==
  GM : Inport
  Scope : Scope
  Scope1 : Scope
  Sum1 : Sum  Inputs=|++
  Uniform Random Number : UniformRandomNumber  Minimum=noise_min  Maximum=noise_max  Seed=noise_seed  SampleTime=lp_sample_time
  noise_k : Gain  Gain=noise_k
  real : Outport
  wires:
  Uniform Random Number/1 -> noise_k/1, Scope1/1
  noise_k/1 -> Scope/1, Sum1/2
  GM/1 -> Sum1/1
  Sum1/1 -> real/1

== system AFCToolbox2023a/SimuMoudle/SimuICM/acclerate  model2/Subsystem1/bias & noise x1 ==
  GM : Inport
  Scope : Scope
  Scope1 : Scope
  Sum1 : Sum  Inputs=|++
  Uniform Random Number : UniformRandomNumber  Minimum=noise_min  Maximum=noise_max  Seed=noise_seed  SampleTime=lp_sample_time
  noise_k : Gain  Gain=noise_k
  real : Outport
  wires:
  Sum1/1 -> real/1
  GM/1 -> Sum1/1
  noise_k/1 -> Sum1/2, Scope/1
  Uniform Random Number/1 -> Scope1/1, noise_k/1

== system AFCToolbox2023a/SimuMoudle/SimuICM/acclerate  model2/Subsystem2/bias & noise x1 ==
  GM : Inport
  Scope : Scope
  Scope1 : Scope
  Sum1 : Sum  Inputs=|++
  Uniform Random Number : UniformRandomNumber  Minimum=noise_min  Maximum=noise_max  Seed=noise_seed  SampleTime=lp_sample_time
  noise_k : Gain  Gain=noise_k
  real : Outport
  wires:
  Uniform Random Number/1 -> noise_k/1, Scope1/1
  noise_k/1 -> Scope/1, Sum1/2
  GM/1 -> Sum1/1
  Sum1/1 -> real/1

== system AFCToolbox2023a/SimuMoudle/SimuICM/gyro model1/Subsystem/bias & noise x1 ==
  GM : Inport
  Scope : Scope
  Scope1 : Scope
  Sum1 : Sum  Inputs=|++
  Uniform Random Number : UniformRandomNumber  Minimum=noise_min  Maximum=noise_max  Seed=noise_seed  SampleTime=lp_sample_time
  noise_k : Gain  Gain=noise_k
  real : Outport
  wires:
  Sum1/1 -> real/1
  GM/1 -> Sum1/1
  noise_k/1 -> Sum1/2, Scope/1
  Uniform Random Number/1 -> Scope1/1, noise_k/1

== system AFCToolbox2023a/SimuMoudle/SimuICM/gyro model1/Subsystem1/bias & noise x1 ==
  GM : Inport
  Scope : Scope
  Scope1 : Scope
  Sum1 : Sum  Inputs=|++
  Uniform Random Number : UniformRandomNumber  Minimum=noise_min  Maximum=noise_max  Seed=noise_seed  SampleTime=lp_sample_time
  noise_k : Gain  Gain=noise_k
  real : Outport
  wires:
  Uniform Random Number/1 -> noise_k/1, Scope1/1
  noise_k/1 -> Scope/1, Sum1/2
  GM/1 -> Sum1/1
  Sum1/1 -> real/1

== system AFCToolbox2023a/SimuMoudle/SimuICM/gyro model1/Subsystem2/bias & noise x1 ==
  GM : Inport
  Scope : Scope
  Scope1 : Scope
  Sum1 : Sum  Inputs=|++
  Uniform Random Number : UniformRandomNumber  Minimum=noise_min  Maximum=noise_max  Seed=noise_seed  SampleTime=lp_sample_time
  noise_k : Gain  Gain=noise_k
  real : Outport
  wires:
  Sum1/1 -> real/1
  GM/1 -> Sum1/1
  noise_k/1 -> Sum1/2, Scope/1
  Uniform Random Number/1 -> Scope1/1, noise_k/1

== system AFCToolbox2023a/SimuMoudle/UAV/Forces & Moments/Forces/Subsystem ==
  Zero : Inport
  g0 : Inport  Port=2
  Mux1 : Mux  Inputs=3
  gravity : Outport
  wires:
  Zero/1 -> Mux1/2, Mux1/1
  Mux1/1 -> gravity/1
  g0/1 -> Mux1/3

== system AFCToolbox2023a/SimuMoudle/UAV/Forces & Moments/Moments/Disturb ==
  Moment : Inport
  Demux : Demux  Outputs=3
  Dist Mx : Subsystem  mask(Step Disturbe){ts_0=lp_momentx_ts, A0=lp_momentx_A0, Af=lp_momentx_Af}
      mask prompts: ts_0 "Step time (s) :"; A0 "Initial Value (N.m) :"; Af "Final Value (N.m) :"
  Dist My : Subsystem  mask(Step Disturbe){ts_0=lp_momenty_ts, A0=lp_momenty_A0, Af=lp_momenty_Af}
      mask prompts: ts_0 "Step time (s) :"; A0 "Initial Value (N.m) :"; Af "Final Value (N.m) :"
  Dist Mz : Subsystem  mask(Step Disturbe){ts_0=lp_momentz_ts, A0=lp_momentz_A0, Af=lp_momentz_Af}
      mask prompts: ts_0 "Step time (s) :"; A0 "Initial Value (N.m) :"; Af "Final Value (N.m) :"
  Mux : Mux  Inputs=3
  M : Outport
  wires:
  Mux/1 -> M/1
  Moment/1 -> Demux/1
  Demux/1 -> Dist Mx/1(N)
  Demux/2 -> Dist My/1(N)
  Demux/3 -> Dist Mz/1(N)
  Dist Mx/1(D) -> Mux/1
  Dist My/1(D) -> Mux/2
  Dist Mz/1(D) -> Mux/3

== system AFCToolbox2023a/SimuMoudle/UAV/Forces & Moments/Parameters/Air Parameter1 ==
  V : Inport
  h(m) : Inport  Port=2
  Air Model : Subsystem
  Fcn : Fcn  Expr=g0*(6371^2/(6371+u)^2)
  Gain3 : Gain  Gain=0.001
  vel : Scope
  Mach : Outport
  q : Outport  Port=2
  Pressure : Outport  Port=3
  g : Outport  Port=4
  wires:
  Air Model/3(Pressure) -> Pressure/1
  Gain3/1 -> Fcn/1, Air Model/2(h (km))
  Air Model/1(dongYaTou) -> q/1
  Air Model/2(Mach) -> Mach/1
  V/1 -> vel/1, Air Model/1(v)
  h(m)/1 -> Gain3/1
  Fcn/1 -> g/1

== system AFCToolbox2023a/SimuMoudle/UAV/Forces & Moments/Parameters/Inertia Solution ==
  Constant : Constant  Value=I_xyz
  lp_kIxyz : Gain  Gain=lp_kIxyz
  Inertia : Outport
  wires:
  Constant/1 -> lp_kIxyz/1
  lp_kIxyz/1 -> Inertia/1

== system AFCToolbox2023a/SimuMoudle/UAV/Forces & Moments/Parameters/Wind Velocity ==
  height : Inport
  >lp_hf_vwind : Switch  Criteria=u2 > Threshold  Threshold=lp_hf_vwind  SaturateOnIntegerOverflow=off  InputSameDT=off
  Lookup Table h-v wind : Lookup  InputValues=lp_hs_vwind_interp  Table=lp_vs_vwind_interp  SaturateOnIntegerOverflow=off
  Vector : Subsystem
  lp_vf_vwind : Constant  Value=lp_vf_vwind
  lp_vwind_thetax : Constant  Value=lp_vwind_thetax
  lp_vwind_thetaz : Constant  Value=lp_vwind_thetaz
  V Wind : Outport
  wires:
  lp_vf_vwind/1 -> >lp_hf_vwind/1
  height/1 -> Lookup Table h-v wind/1, >lp_hf_vwind/2
  Lookup Table h-v wind/1 -> >lp_hf_vwind/3
  lp_vwind_thetaz/1 -> Vector/2(thetaz)
  lp_vwind_thetax/1 -> Vector/3(thetax)
  Vector/1(xyz) -> V Wind/1
  >lp_hf_vwind/1 -> Vector/1(abs)

== system AFCToolbox2023a/SimuMoudle/UAV/Forces & Moments/Parameters/mass P ==
  Constant 1 : Constant  Value=mass
  lp_kmass : Gain  Gain=lp_kmass
  mass : Outport
  wires:
  lp_kmass/1 -> mass/1
  Constant 1/1 -> lp_kmass/1

== system AFCToolbox2023a/SimuMoudle/UAV/Forces & Moments/Parameters/modulus of vector ==
  vector : Inport
  Divide2 : Product
  Math Function : Math  Operator=sqrt  SignedPower=on
  Sum of Elements : Sum  Inputs=+
  modulus : Outport
  wires:
  Math Function/1 -> modulus/1
  vector/1 -> Divide2/1, Divide2/2
  Divide2/1 -> Sum of Elements/1
  Sum of Elements/1 -> Math Function/1

== system AFCToolbox2023a/基础导航算法模型库/ECL EKF/Subsystem/GPS Fusion1/Control BARO_Hgt Fusion ==
  "states " : Inport
  "P " : Inport  Port=2
  meas_Hgt : Inport  Port=3
  baro_hgt_offset : Inport  Port=4
  Control Baro_Height Fusion1 : MATLAB Function  TreatAsAtomicUnit=on
  Terminator4 : Terminator
  Terminator5 : Terminator
  obs_var_baro : Constant  Value=obs_var_baro
  states : Outport
  P : Outport  Port=2
  wires:
  obs_var_baro/1 -> Control Baro_Height Fusion1/6(params_baro_noise)
  Control Baro_Height Fusion1/4(innov_var) -> Terminator4/1
  Control Baro_Height Fusion1/3(innovation) -> Terminator5/1
  meas_Hgt/1 -> Control Baro_Height Fusion1/3(measHgt)
  Control Baro_Height Fusion1/1(states) -> states/1
  "states "/1 -> Control Baro_Height Fusion1/1("states ")
  Control Baro_Height Fusion1/2(P) -> P/1
  baro_hgt_offset/1 -> ?
  "P "/1 -> Control Baro_Height Fusion1/2("P ")

== system AFCToolbox2023a/基础导航算法模型库/ECL EKF/init_state/ALIGN TILT 1/Subsystem ==
  init_quat : Inport
  initAccel : Inport  Port=2
  Atan2 : Trigonometry  Operator=atan2
  Constant : Constant  Value=[0,0,-1]  OutDataTypeStr=single
  Cross Product : matrix_library/Cross Product
  Divide : Product  Inputs=*/
  Divide1 : Product  Inputs=*/
  Dot Product : DotProduct  OutDataTypeStr=Inherit: Inherit via internal rule
  Dot Product1 : DotProduct  OutDataTypeStr=Inherit: Inherit via internal rule
  Gain : Gain  Gain=-1
  Gain1 : Gain  Gain=0.5
  Gain2 : Gain  Gain=0.5
  Mux : Mux  Inputs=2
  Product : Product
  Product1 : Product
  Reshape : Reshape  OutputDimensionality=Customize  OutputDimensions=[4,1]
  Selector : Selector  InputPortWidth=3  IndexOptions=Index vector (dialog)  Indices=[1 2]  OutputSizes=1
  Selector1 : Selector  InputPortWidth=3  IndexOptions=Index vector (dialog)  Indices=[3]  OutputSizes=1
  Sqrt : Sqrt
  Sqrt1 : Sqrt
  Switch3 : Switch  Criteria=u2 > Threshold  Threshold=0.001  SaturateOnIntegerOverflow=off  InputSameDT=off
  Trigonometric Function : Trigonometry  Operator=cos
  Trigonometric Function1 : Trigonometry
  quat : Outport
  wires:
  Switch3/1 -> quat/1
  init_quat/1 -> Switch3/3
  initAccel/1 -> Cross Product/1, Selector1/1, Selector/1
  Dot Product/1 -> Sqrt/1
  Selector/1 -> Dot Product/1, Dot Product/2
  Sqrt/1 -> Atan2/1
  Selector1/1 -> Gain/1
  Gain/1 -> Atan2/2
  Atan2/1 -> Product/2, Divide1/2, Switch3/2, Gain2/1, Gain1/1
  Constant/1 -> Cross Product/2
  Cross Product/1 -> Divide/1, Dot Product1/2, Dot Product1/1
  Dot Product1/1 -> Sqrt1/1
  Sqrt1/1 -> Divide/2
  Gain1/1 -> Trigonometric Function/1
  Trigonometric Function1/1 -> Product1/2
  Gain2/1 -> Trigonometric Function1/1
  Product1/1 -> Mux/2
  Trigonometric Function/1 -> Mux/1
  Divide/1 -> Product/1
  Product/1 -> Divide1/1
  Divide1/1 -> Product1/1
  Mux/1 -> Reshape/1
  Reshape/1 -> Switch3/1

== system AFCToolbox2023a/基础导航算法模型库/ECL EKF/init_state/InitState_accel1/Subsystem ==
  data : Inport
  Buffer : Buffer  N=99  V=98  OutputFrames=off
  Buffer1 : Buffer  N=99  V=98  OutputFrames=off
  Buffer2 : Buffer  N=99  V=98  OutputFrames=off
  Demux : Demux  Outputs=3
  Mean4 : dspstat3/Mean  run=off  reset_popup=None  directionMode=Entire input  dimension=3  roiEnable=off  roiType=Rectangles  roiPortion=Entire ROI  roiOutput=Individual statistics for each ROI  roiFlag=off  roundingMode=Floor  overflowMode=off  outputDataTypeStr=Inherit: Same as accumulator  outputMin=[]  outputMax=[]  outputLastDataTypeStr=Inherit: Same as accumulator
  Mean5 : dspstat3/Mean  run=off  reset_popup=None  directionMode=Entire input  dimension=3  roiEnable=off  roiType=Rectangles  roiPortion=Entire ROI  roiOutput=Individual statistics for each ROI  roiFlag=off  roundingMode=Floor  overflowMode=off  outputDataTypeStr=Inherit: Same as accumulator  outputMin=[]  outputMax=[]  outputLastDataTypeStr=Inherit: Same as accumulator
  Mean6 : dspstat3/Mean  run=off  reset_popup=None  directionMode=Entire input  dimension=3  roiEnable=off  roiType=Rectangles  roiPortion=Entire ROI  roiOutput=Individual statistics for each ROI  roiFlag=off  roundingMode=Floor  overflowMode=off  outputDataTypeStr=Inherit: Same as accumulator  outputMin=[]  outputMax=[]  outputLastDataTypeStr=Inherit: Same as accumulator
  Scope : Scope  NumInputPorts=2
  Vector Concatenate : Concatenate  NumInputs=3
  mean_data : Outport
  wires:
  Mean6/1 -> Vector Concatenate/3
  Demux/2 -> Buffer1/1
  Buffer/1 -> Mean4/1  "fbx_buff"
  Mean5/1 -> Vector Concatenate/2
  Buffer2/1 -> Mean6/1  "fbz_buff"
  Demux/1 -> Buffer/1
  Buffer1/1 -> Mean5/1  "fby_buff"
  Demux/3 -> Buffer2/1
  Mean4/1 -> Vector Concatenate/1
  Vector Concatenate/1 -> Scope/2, mean_data/1
  data/1 -> Scope/1, Demux/1

== system AFCToolbox2023a/基础导航算法模型库/ECL EKF/init_state/InitState_baro1/TD_baro ==
  H_baro : Inport
  Constant1 : Constant  Value=dt  OutDataTypeStr=single
  Constant3 : Constant  Value=0.23  OutDataTypeStr=single
  Constant4 : Constant  Value=900  OutDataTypeStr=single
  Data Type Conversion5 : DataTypeConversion  OutDataTypeStr=single  SaturateOnIntegerOverflow=off  RndMeth=Floor
  Delay1 : Delay  DelayLength=1  InitialConditionSource=Input port
      settings: InputPortMap=u0,p4
  MATLAB Function2 : MATLAB Function  TreatAsAtomicUnit=on
  Memory : Memory  InheritSampleTime=on
  Scope : Scope  NumInputPorts=3
  vH_baro_TD : Outport
  H_baro_TD : Outport  Port=2
  wires:
  Delay1/1 -> H_baro_TD/1, Scope/3, MATLAB Function2/3("u1 ")
  H_baro/1 -> Data Type Conversion5/1
  Memory/1 -> MATLAB Function2/4("u2 "), vH_baro_TD/1, Scope/2
  Constant3/1 -> MATLAB Function2/5(h)
  Constant1/1 -> MATLAB Function2/1(T)
  Constant4/1 -> MATLAB Function2/6(r)
  MATLAB Function2/1(u1) -> Delay1/1
  MATLAB Function2/2(u2) -> Memory/1
  Data Type Conversion5/1 -> Scope/1, Delay1/2, MATLAB Function2/2(u0)

== system AFCToolbox2023a/基础导航算法模型库/ECL EKF/init_state/InitState_baro1/reinit_baro0 ==
  Data : Inport
  QGC_sensor_reinit : Inport  Port=2
  Detect Increase : simulink/Logic and Bit Operations/Detect Increase  vinit=0.0  OutDataTypeStr=boolean
  Switch : Switch  Criteria=u2 > Threshold  SaturateOnIntegerOverflow=off  InputSameDT=off
  Unit Delay : UnitDelay  SampleTime=-1  HasFrameUpgradeWarning=on
  dataout : Outport
  wires:
  Unit Delay/1 -> Switch/3
  Data/1 -> Switch/1
  Switch/1 -> dataout/1, Unit Delay/1
  Detect Increase/1 -> Switch/2
  QGC_sensor_reinit/1 -> Detect Increase/1

== system AFCToolbox2023a/基础导航算法模型库/ECL EKF/init_state/State_mag1/Subsystem ==
  data : Inport
  Buffer : Buffer  N=9  V=8  OutputFrames=off
  Buffer1 : Buffer  N=9  V=8  OutputFrames=off
  Buffer2 : Buffer  N=9  V=8  OutputFrames=off
  Demux : Demux  Outputs=3
  Mean4 : dspstat3/Mean  run=off  reset_popup=None  directionMode=Entire input  dimension=3  roiEnable=off  roiType=Rectangles  roiPortion=Entire ROI  roiOutput=Individual statistics for each ROI  roiFlag=off  roundingMode=Floor  overflowMode=off  outputDataTypeStr=Inherit: Same as accumulator  outputMin=[]  outputMax=[]  outputLastDataTypeStr=Inherit: Same as accumulator
  Mean5 : dspstat3/Mean  run=off  reset_popup=None  directionMode=Entire input  dimension=3  roiEnable=off  roiType=Rectangles  roiPortion=Entire ROI  roiOutput=Individual statistics for each ROI  roiFlag=off  roundingMode=Floor  overflowMode=off  outputDataTypeStr=Inherit: Same as accumulator  outputMin=[]  outputMax=[]  outputLastDataTypeStr=Inherit: Same as accumulator
  Mean6 : dspstat3/Mean  run=off  reset_popup=None  directionMode=Entire input  dimension=3  roiEnable=off  roiType=Rectangles  roiPortion=Entire ROI  roiOutput=Individual statistics for each ROI  roiFlag=off  roundingMode=Floor  overflowMode=off  outputDataTypeStr=Inherit: Same as accumulator  outputMin=[]  outputMax=[]  outputLastDataTypeStr=Inherit: Same as accumulator
  Vector Concatenate : Concatenate  NumInputs=3
  mean_data : Outport
  wires:
  data/1 -> Demux/1
  Vector Concatenate/1 -> mean_data/1
  Mean4/1 -> Vector Concatenate/1
  Demux/3 -> Buffer2/1
  Buffer1/1 -> Mean5/1  "fby_buff"
  Demux/1 -> Buffer/1
  Buffer2/1 -> Mean6/1  "fbz_buff"
  Mean5/1 -> Vector Concatenate/2
  Buffer/1 -> Mean4/1  "fbx_buff"
  Demux/2 -> Buffer1/1
  Mean6/1 -> Vector Concatenate/3

== system AFCToolbox2023a/基础导航算法模型库/ECL EKF/init_state/State_mag1/Subsystem1 ==
  note: % EKF2.cpp -> UpdateGpsSample(...) ->
      | ~ estimator.cpp ->  setGpsData(..) ->
      | ~ gps_checks.cpp -> get_mag_declination_radians(...) -> get_mag_inclination_radians(...) -> get_mag_strength_gauss(...)
  lat_rad : Inport
  lon_rad : Inport  Port=2
  Display : Display
  Display1 : Display
  Display2 : Display
  Gain : Gain  Gain=57.3
  Gain1 : Gain  Gain=57.3
  Gain2 : Gain  Gain=57.3
  Scope : Scope
  Subsystem : Subsystem
  Subsystem2 : Subsystem
  Subsystem3 : Subsystem
  mag_declination_gps : Outport  VectorParamsAs1DForOutWhenUnconnected=off
  mag_inclination_gps : Outport  Port=2  VectorParamsAs1DForOutWhenUnconnected=off
  mag_strength_gps : Outport  Port=3  VectorParamsAs1DForOutWhenUnconnected=off
  wires:
  Subsystem/1(get_mag_declination_rad) -> Gain/1, mag_declination_gps/1
  lat_rad/1 -> Scope/1, Subsystem/1(lat_rad), Subsystem2/1(lat_rad), Subsystem3/1(lat_rad)
  lon_rad/1 -> Subsystem2/2(lon_rad), Subsystem3/2(lon_rad), Subsystem/2(lon_rad)
  Subsystem3/1(get_mag_inclination_rad) -> Gain1/1, mag_inclination_gps/1
  Subsystem2/1(get_mag_strength_gauss) -> Gain2/1, mag_strength_gps/1
  Gain/1 -> Display/1
  Gain1/1 -> Display1/1
  Gain2/1 -> Display2/1

== system AFCToolbox2023a/基础导航算法模型库/ECL EKF/init_state/State_mag1/calculate_synthetic_mag_z_measurement ==
  note: % ~ mag_control.cpp -> controlMagFusion(...) ->
      | ~ mag_fusion.cpp -> calculate_synthetic_mag_z_measurement(...)
  measMag : Inport
  _mag_declination_gps : Inport  Port=2
  _mag_inclination_gps : Inport  Port=3
  _mag_strength_gps : Inport  Port=4
  _R_to_earth : Inport  Port=5
  Constant1 : Constant  Value=0
  Constant2 : Constant  Value=0
  Constant3 : Constant  Value=0
  Demux1 : Demux  Outputs=3
  Dot Product : DotProduct  OutDataTypeStr=Inherit: Inherit via internal rule
  Dot Product1 : DotProduct  OutDataTypeStr=Inherit: Inherit via internal rule
  Gain : Gain  Gain=-1
  Gain1 : Gain  Gain=-1
  Max : MinMax  Function=max  Inputs=2
  Mux : Mux  Inputs=3
  Mux1 : Mux  Inputs=3
  Product : Product  Multiplication=Matrix(*)
  Rotation Angles to Direction Cosine Matrix : sharedtransform/Rotation Angles to Direction Cosine Matrix  rotationOrder=ZYX  aMode=aMode
  Scope : Scope
  Scope1 : Scope
  Selector : Selector  InputPortWidth=3  IndexOptions=Index vector (dialog)  Indices=1  OutputSizes=1
  Selector1 : Selector  NumberOfDimensions=2  InputPortWidth=3  IndexOptions=Index vector (dialog),Index vector (dialog)  Indices=[1:3],[3]  OutputSizes=1,1
  Sqrt : Sqrt
  Sqrt1 : Sqrt
  Square : Math  Operator=square
  Square1 : Math  Operator=square
  Square2 : Math  Operator=square
  Subtract : Sum  Inputs=--+
  Sum of Elements : Sum  Inputs=+
  Switch2 : Switch  Criteria=u2 > Threshold  SaturateOnIntegerOverflow=off  InputSameDT=off
  Terminator2 : Terminator
  mag_z_body_pred : Outport
  wires:
  Sqrt1/1 -> Gain1/1, Switch2/1  "mag_z_abs"
  Product/1 -> Selector/1, Scope1/1, Dot Product/1, Dot Product/2  "mag_earth_pred"
  Constant2/1 -> Mux1/3, Mux1/2
  Demux1/2 -> Square1/1
  Constant1/1 -> Mux/3
  Switch2/1 -> mag_z_body_pred/1
  Mux/1 -> Rotation Angles to Direction Cosine Matrix/1
  Dot Product1/1 -> Scope/1
  Subtract/1 -> Max/2
  Demux1/3 -> Terminator2/1
  _R_to_earth/1 -> Selector1/1
  Max/1 -> Sqrt1/1
  _mag_strength_gps/1 -> Mux1/1
  Square/1 -> Subtract/1
  Constant3/1 -> Max/1
  Sum of Elements/1 -> Sqrt/1
  Square1/1 -> Subtract/2
  Sqrt/1 -> Square2/1
  Mux1/1 -> Product/2
  Gain/1 -> Mux/2
  Demux1/1 -> Square/1
  Rotation Angles to Direction Cosine Matrix/1 -> Product/1
  measMag/1 -> Demux1/1
  Gain1/1 -> Switch2/3
  _mag_inclination_gps/1 -> Gain/1
  _mag_declination_gps/1 -> Mux/1
  Selector1/1 -> Dot Product1/2
  Square2/1 -> Subtract/3
  Dot Product/1 -> Sum of Elements/1
  Selector/1 -> Switch2/2

== system AFCToolbox2023a/基础导航算法模型库/ECL EKF/init_state/State_mag1/mag_lpf ==
  Mag_Data : Inport
  Add : Sum
  Delay : Delay  DelayLength=1  InitialConditionSource=Input port  InitialCondition=0  ExternalReset=Rising  UseCircularBuffer=on
      settings: InputPortMap=u0,r5,p4
  Detect Increase : simulink/Logic and Bit Operations/Detect Increase  vinit=0.0  OutDataTypeStr=boolean
  Detect Increase1 : simulink/Logic and Bit Operations/Detect Increase  vinit=0.0  OutDataTypeStr=boolean
  Gain : Gain  Gain=0.1
  Gain1 : Gain  Gain=0.9
  Scope : Scope
  Selector : Selector  InputPortWidth=3  IndexOptions=Index vector (dialog)  Indices=[1]  OutputSizes=1
  Switch : Switch  Criteria=u2 > Threshold  SaturateOnIntegerOverflow=off  InputSameDT=off
  Unit Delay : UnitDelay  SampleTime=-1  HasFrameUpgradeWarning=on
  mag_lpf : Outport
  wires:
  Unit Delay/1 -> Switch/3
  Mag_Data/1 -> Detect Increase/1, Switch/1
  Switch/1 -> Selector/1, Unit Delay/1, Delay/3, Gain/1
  Detect Increase/1 -> Switch/2
  Gain/1 -> Add/1
  Gain1/1 -> Add/2
  Delay/1 -> Gain1/1, Scope/1, mag_lpf/1
  Add/1 -> Delay/1
  Detect Increase1/1 -> Delay/2
  Selector/1 -> Detect Increase1/1

== system AFCToolbox2023a/SimuMoudle/Forces & Moments1/Parameters/Air Parameter1/Air Model/H ==
  h : Inport
  1 : Constant
  Add1 : Sum  Inputs=2
  Product4 : Product  Inputs=*/  RndMeth=Zero
  Product5 : Product  Inputs=*/  RndMeth=Zero
  R0 : Constant  Value=6356.766
  H : Outport
  wires:
  Product5/1 -> H/1
  Add1/1 -> Product5/2
  1/1 -> Add1/2
  Product4/1 -> Add1/1
  R0/1 -> Product4/2
  h/1 -> Product5/1, Product4/1
